simulink model "currentModelSPM"  (R2025a)
settings: Solver=VariableStepAuto  StartTime=0.0  StopTime=4500  RelTol=1e-3
libraries: fl_lib x8, nesl_utility x6, BatteryCurrentManagement x2, batt_lib x1, BatteryEstimators x1
settings Model: Creator=rdsti  LastModifiedBy=rdsti

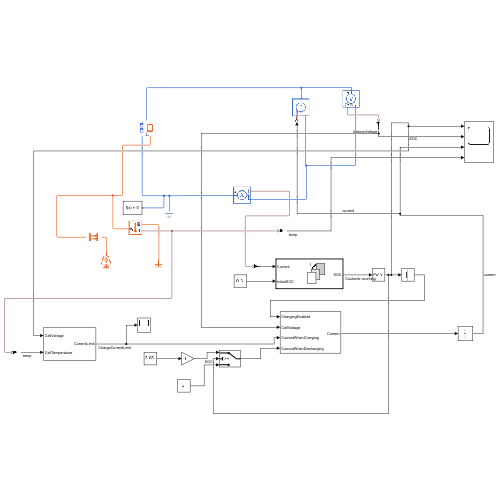
[thumbnail: Simulink's stored preview of the top-level diagram]
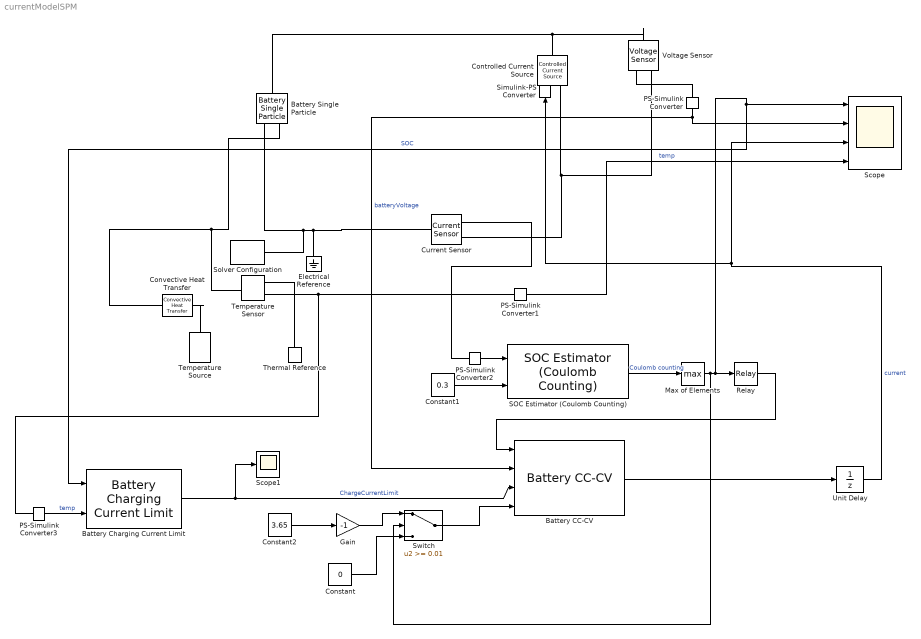
== system currentModelSPM ==
  Battery CC-CV : BatteryCurrentManagement/Battery CC-CV  MinMaxFlag=off  MaxCellVoltage=4  Kp=100  Ki=10  Kaw=1  Kt=1  Ts=-1
      settings: LibrarySourceBlock=batt_sl_lib/Current Management/Battery CC-CV
  Battery Charging Current Limit : BatteryCurrentManagement/Battery Charging Current Limit  MinMaxFlag=off  CellOvervoltageLimit=4.48  R0=0.0025  T_vec=[243.15, 258.15, 273.15, 288.15, 303.15, 318.15, 333.15]  CurrentLimitCoolestCell=[ 0, 0, 0, 0, 100, 100, 100]  CurrentLimitHottestCell=[100, 100, 100, 100, 0, 0, 0]  DataType=Inherit: auto
      settings: LibrarySourceBlock=|
      | batt_sl_lib/Current Management/Battery Charging
      | Current Limit
  Battery Single Particle : batt_lib/Cells/Electrochemical/Battery Single Particle  ExtrapolationMethod=simscape.enum.extrapolation.nearest  ThicknessAnode=3.4E-5 m  ElectrolyteLayerCountAnode=10  ThicknessSeparator=2.5E-5 m  ElectrolyteLayerCountSeparator=5  ThicknessCathode=8E-5 m  ElectrolyteLayerCountCathode=10  ElectrodePlateArea=1.8E-1 m^2  ParticleRadiusAnode=5E-6 m  ShellCountAnode=10  ParticleRadiusCathode=5E-8 m  ShellCountCathode=10  ActiveMaterialVolumeFractionAnode=0.58  ActiveMaterialVolumeFractionCathode=0.374  StoichiometryBreakpointsSpecification=simscape.battery.enum.cells.electrochemical.StoichiometryBreakpointsSpecification.normalized  NormalizedStoichiometryBreakpoints=linspace(0.025, 0.975, 39)  OpenCircuitPotentialAnode=[.435; .325; .259; .221; .204; .194; .179; .166; .155; .145; .137; .131; .128; .127; .126; .125; .124; .123; .122; .121; .118; .117; .112; .109; .105; .1; .098; .095; .094; .093; .091; .09; .089; .088; .087; .086; .085; .084; .083] V  OpenCircuitPotentialCathode=[3.598; 3.53; 3.494; 3.474; 3.46; 3.455; 3.454; 3.453; 3.4528; 3.4526; 3.4524; 3.452; 3.4518; 3.4516; 3.4514; 3.4512; 3.451; 3.4508; 3.4506; 3.4503; 3.45; 3.4498; 3.4495; 3.4493; 3.449; 3.4488; 3.4486; 3.4484; 3.4482; 3.4479; 3.4477; 3.4475; 3.4473; 3.447; 3.4468; 3.4466; 3.4464; 3.4462; 3.4458] V  AbsoluteStoichiometryBreakpointsAnode=linspace(0.025, 0.975, 39)  OpenCircuitPotentialAbsoluteAnode=[.484; .335; .253; .209; .2; .181; .165; .151; .139; .131; .128; .125; .124; .124; .123; .122; .119; .117; .111; .108; .101; .098; .095; .093; .092; .088; .088; .088; .088; .087; .087; .087; .085; .082; .079; .071; .064; .049; .026] V  AbsoluteStoichiometryBreakpointsCathode=linspace(0.025, 0.975, 39)  OpenCircuitPotentialAbsoluteCathode=[3.81; 3.608; 3.512; 3.478; 3.459; 3.453; 3.45257; 3.45214; 3.45171; 3.45128; 3.45085; 3.45042; 3.44999; 3.44956; 3.44913; 3.4487; 3.44827; 3.44784; 3.44741; 3.44698; 3.44655; 3.44612; 3.44569; 3.44526; 3.44483; 3.4444; 3.44397; 3.44354; 3.44311; 3.44268; 3.44225; 3.44182; 3.44139; 3.44096; 3.44053; 3.44; 3.412; 3.304; 2.968] V  MaximumConcentrationAnode=30555 mol/m^3  MaximumStoichiometryAnode=0.811  MinimumStoichiometryAnode=0.0132  MaximumConcentrationCathode=22806 mol/m^3  MaximumStoichiometryCathode=0.74  MinimumStoichiometryCathode=0.035  ActiveMaterialDiffusionCoefficientAnode=3E-15 m^2/s  ActiveMaterialDiffusionCoefficientCathode=5.9E-20 m^2/s  ConductivityAnode=100 S/m  ConductivityCathode=0.5 S/m  CurrentCollectorResistance=0 Ohm  ElectrolyteVolumeFractionAnode=0.3874  ElectrolyteVolumeFractionSeparator=0.45  ElectrolyteVolumeFractionCathode=0.5725  ElectrolyteConductivity=0.29 S/m  BruggemanExponentAnode=1.5  BruggemanExponentSeparator=1.5  BruggemanExponentCathode=1.5  TransferenceNumber=0.363  ElectrolyteDiffusionCoefficient=2E-10 m^2/s  ChargeTransferRateAnode=8.8E-11 m^(5/2)/(mol^(1/2)*s)  ChargeTransferRateCathode=2.8E-13 m^(5/2)/(mol^(1/2)*s)  BatteryThermalMass=77 J/K  ArrheniusReferenceTemperature=298.15 K  ActiveMaterialDiffusionActivationEnergyAnode=39000 J/mol  ActiveMaterialDiffusionActivationEnergyCathode=35000 J/mol  ElectrolyteDiffusionActivationEnergy=26600 J/mol  ConductivityActivationEnergyAnode=3000 J/mol  ConductivityActivationEnergyCathode=3000 J/mol  ElectrolyteConductivityActivationEnergy=11000 J/mol  ChargeTransferActivationEnergyAnode=13000 J/mol  ChargeTransferActivationEnergyCathode=20000 J/mol  batteryCurrent_specify=off  batteryCurrent_priority=None  batteryCurrent=0 A  batteryCurrent_nominal_specify=off  batteryCurrent_nominal_value=1  batteryCurrent_nominal_unit=A  batteryVoltage_specify=off  batteryVoltage_priority=None  batteryVoltage=0 V  batteryVoltage_nominal_specify=off  batteryVoltage_nominal_value=1  batteryVoltage_nominal_unit=V  averageElectrolyteConcentration_specify=off  averageElectrolyteConcentration_priority=High  averageElectrolyteConcentration=1200 mol/m^3  averageElectrolyteConcentration_nominal_specify=off  averageElectrolyteConcentration_nominal_value=1  averageElectrolyteConcentration_nominal_unit=mol/m^3  stateOfCharge_specify=on  stateOfCharge_priority=High  stateOfCharge=0.3  stateOfCharge_nominal_specify=off  stateOfCharge_nominal_value=1  stateOfCharge_nominal_unit=1  batteryTemperature_specify=off  batteryTemperature_priority=High  batteryTemperature=298.15 K  batteryTemperature_nominal_specify=off  batteryTemperature_nominal_value=1  batteryTemperature_nominal_unit=K  power_dissipated_specify=off  power_dissipated_priority=None  power_dissipated=0 W  power_dissipated_nominal_specify=off  power_dissipated_nominal_value=1  power_dissipated_nominal_unit=W  heatGenerationRate_specify=off  heatGenerationRate_priority=None  heatGenerationRate=0 W  heatGenerationRate_nominal_specify=off  heatGenerationRate_nominal_value=1  heatGenerationRate_nominal_unit=W
      settings: InternalSimscapePortConfiguration="{\"Bottom\":[],\"Left\":[{\"id\":\"p\",\"label\":\"+\",\"type\":\"foundation.electrical.electrical\"}],\"Right\":[{\"id\":\"n\",\"label\":\"-\",\"type\":\"foundation.electrical.electrical\"},{\"id\":\"H\",\"label\":\"H\",\"type\":\"foundation.thermal.thermal\"}],\"Top\":[]}"
  Constant : Constant  Value=0
  Constant1 : Constant  Value=0.3
  Constant2 : Constant  Value=3.65
  Controlled Current Source : fl_lib/Electrical/Electrical Sources/Controlled Current Source
  Convective Heat Transfer : fl_lib/Thermal/Thermal Elements/Convective Heat Transfer  thermal_type=foundation.enum.constant_variable.constant  area=0.0034 m^2  heat_tr_coeff=10 W/(K*m^2)  min_heat_tr_coeff=1e-3 W/(K*m^2)  T_specify=off  T_priority=None  T=0 K  T_nominal_specify=off  T_nominal_value=1  T_nominal_unit=K  Q_specify=off  Q_priority=None  Q=0 W  Q_nominal_specify=off  Q_nominal_value=1  Q_nominal_unit=W
  Current Sensor : fl_lib/Electrical/Electrical Sensors/Current Sensor
  Electrical Reference : fl_lib/Electrical/Electrical Elements/Electrical Reference
  Gain : Gain  Gain=-1
  Max of Elements : MinMax  Function=max
  PS-Simulink Converter{,1..3} (4 alike) : nesl_utility/PS-Simulink Converter  PhysicalDomain=network_engine_domain  SubClassName=ps_output  LeftPortType=input  RightPortType=output  PseudoPeriodic=off  Frequencies=[]  VectorFormat=inherit  Unit=inherit  AffineConversion=off
  Relay : Relay  OnSwitchValue=0.679  OffSwitchValue=0.01  OnOutputValue=0  OffOutputValue=1
  SOC Estimator (Coulomb Counting) : BatteryEstimators/SOC Estimator (Coulomb Counting)  CurrentInputPartition=on  AH=3.349  Ts=1  DataType=Inherit: auto
      settings: LibrarySourceBlock=|
      | batt_sl_lib/Estimators/SOC Estimator
      | (Coulomb Counting)
  Scope : Scope  NumInputPorts=4
      settings: ActiveDisplayYMinimum=0.24209090617171142  ActiveDisplayYMaximum=0.72761622882190424
  Scope1 : Scope
      settings: ActiveDisplayYMinimum=-3.085534851193283  ActiveDisplayYMaximum=37.379874242725194
  Simulink-PS Converter : nesl_utility/Simulink-PS Converter  PhysicalDomain=network_engine_domain  SubClassName=ps_input  LeftPortType=input  RightPortType=output  PseudoPeriodic=off  Frequencies=[]  NoiseDistribution=none  NoiseParameters=[]  Unit=1  AffineConversion=off  FilteringAndDerivatives=provide  SimscapeFilterOrder=1  InputFilterTimeConstant=0.001  UdotUserProvided=0
  Solver Configuration : nesl_utility/Solver Configuration  PhysicalDomain=network_engine_domain  SubClassName=solver  LeftPortType=input  RightPortType=generic  Tones=[]  Harmonics=[]  SimulateNoise=off  Profile=off  UseLocalSampling=off  EnableSwitchedLinearOptims=on  FrequencyDomain=off  UseCCode=off  RelTol=0.001  AbsTol=0.001  MinStep=1e-09  ToWorkspace=off  RevertToSquareIcSolve=off  NumHomotopyIterations=100  PhasorMode=off  PhasorModeNumHarmonics=1  ConsistencySolver=NEWTON_XTOL_AFTER_FTOL  IndexReductionMethod=DerivativeReplacement  DoDC=off  ResidualTolerance=1e-09  ConsistencyTolSource=GLOBAL  ConsistencyAbsTol=0.001  ConsistencyRelTol=0.001  ConsistencyTolFactor=0.001  UseLocalSolver=off  LocalSolverChoice=NE_BACKWARD_EULER_ADVANCER  ResolveIndetEquations=on  FunctionEvalNumThread=1  LocalSolverSampleTime=0.001  DoFixedCost=off  MaxNonlinIter=3  MaxModeIter=2  ComputeImpulses=off  ImpulseIterations=2  LinearAlgebra=auto  LinearAlgebraNumThread=0  EquationFormulation=NE_TIME_EF  DelaysMemoryBudget=1024  AutomaticFiltering=on  FilteringTimeConstant=0.001  PartitionStorageMethod=AS_NEEDED  PartitionMemoryBudget=1024  PartitionMethod=ROBUST  MultibodyUseLocalSolver=off  MultibodyLocalSolverChoice=ODE1  MultibodyLocalSolverSampleTime=0.001
  Switch : Switch  Threshold=0.01  SaturateOnIntegerOverflow=off  InputSameDT=off
  Temperature Sensor : fl_lib/Thermal/Thermal Sensors/Temperature Sensor  temperature_measure=foundation.enum.MeasurementReference.difference
  Temperature Source : fl_lib/Thermal/Thermal Sources/Temperature Source  temperature=298.15 K
  Thermal Reference : fl_lib/Thermal/Thermal Elements/Thermal Reference
  Unit Delay : UnitDelay  InitialCondition=3.65  SampleTime=-1  HasFrameUpgradeWarning=on
  Voltage Sensor : fl_lib/Electrical/Electrical Sensors/Voltage Sensor
  wires:
  SOC Estimator (Coulomb Counting)/1 -> Max of Elements/1  "Coulomb counting"
  Switch/1 -> Battery CC-CV/4
  Constant2/1 -> Gain/1
  Relay/1 -> Battery CC-CV/1
  Max of Elements/1 -> Switch/2, Battery Charging Current Limit/1, Scope/1, Relay/1  "SOC"
  Constant1/1 -> SOC Estimator (Coulomb Counting)/2
  Gain/1 -> Switch/1
  Constant/1 -> Switch/3
  Unit Delay/1 -> Scope/3, Simulink-PS Converter/1  "current"
  Battery CC-CV/1 -> Unit Delay/1
  PS-Simulink Converter/1 -> Battery CC-CV/2, Scope/2  "batteryVoltage"
  PS-Simulink Converter2/1 -> SOC Estimator (Coulomb Counting)/1
  PS-Simulink Converter3/1 -> Battery Charging Current Limit/2  "temp"
  PS-Simulink Converter1/1 -> Scope/4  "temp"
  Battery Charging Current Limit/1 -> Scope1/1, Battery CC-CV/3  "ChargeCurrentLimit"
  connections:
  Solver Configuration/RConn1 -- Battery Single Particle/RConn1 -- Current Sensor/LConn1 -- Electrical Reference/LConn1
  Convective Heat Transfer/LConn1 -- Battery Single Particle/RConn2 -- Temperature Sensor/LConn1
  Voltage Sensor/LConn1 -- Battery Single Particle/LConn1 -- Controlled Current Source/LConn1
  Simulink-PS Converter/RConn1 -- Controlled Current Source/RConn1
  Temperature Sensor/RConn1 -- Thermal Reference/LConn1
  Convective Heat Transfer/RConn1 -- Temperature Source/LConn1
  PS-Simulink Converter1/LConn1 -- PS-Simulink Converter3/LConn1 -- Temperature Sensor/RConn2
  Voltage Sensor/RConn1 -- PS-Simulink Converter/LConn1
  Voltage Sensor/RConn2 -- Current Sensor/RConn2 -- Controlled Current Source/RConn2
  Current Sensor/RConn1 -- PS-Simulink Converter2/LConn1
